simulink model "Modelado"  (R2023a)
settings: Solver=ode15s  StartTime=0.0  StopTime=15  MaxStep=1E-2  RelTol=1e-3
libraries: fl_lib x7, nesl_utility x3, slpidlib x2
settings Model: Creator=David  LastModifiedBy=David
settings DataIOCC: SaveOutput=off  SignalLogging=off  DSMLogging=off  ReturnWorkspaceOutputs=off  TimeSaveName=t
settings DebuggingCC: AlgebraicLoopMsg=none  ArtificialAlgebraicLoopMsg=none  MaxConsecutiveZCsMsg=none  ModelReferenceExtraNoncontSigs=none  OperatingPointInterfaceChecksumMismatchMsg=none
settings HardwareCC: ProdBitPerPointer=32  ProdBitPerSizeT=32  ProdBitPerPtrDiffT=32  ProdWordSize=32  ProdHWDeviceType=Intel->x86-32 (Windows32)

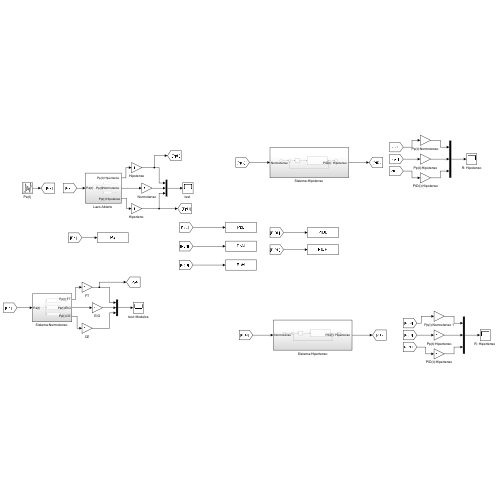
[thumbnail: Simulink's stored preview of the top-level diagram]
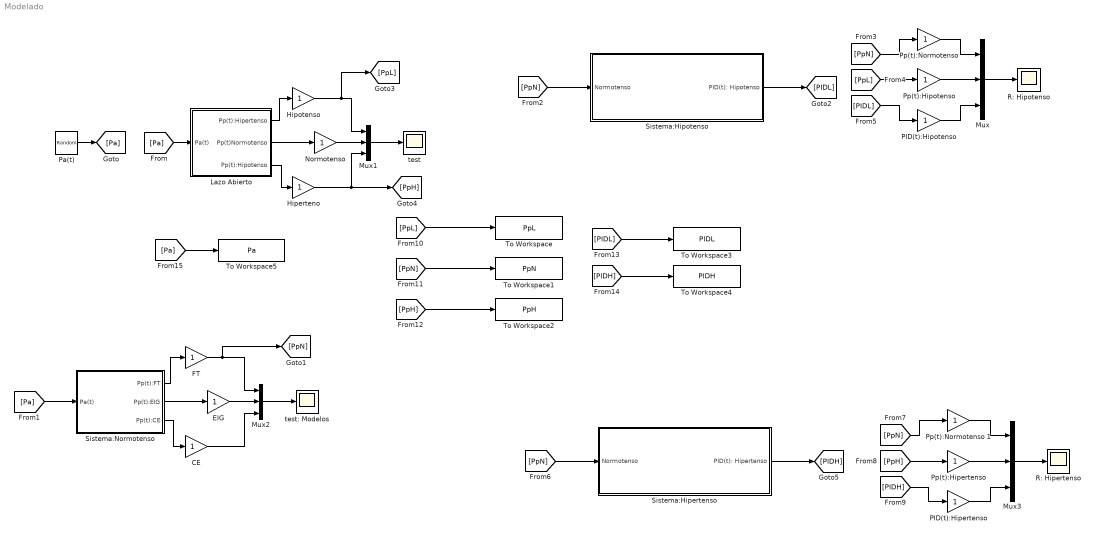
== system Modelado ==
  CE : Gain
  EIG : Gain
  FT : Gain
  "Hiperteno " : Gain
  Hipotenso : Gain
  "Lazo Abierto " : Subsystem
  Mux{,1..3} (4 alike) : Mux  Inputs=3
  Normotenso : Gain
  PID(t):Hipertenso : Gain
  PID(t):Hipotenso : Gain
  Pa(t) : UniformRandomNumber  Minimum=-0.2  Seed=106  SampleTime=0.1
  Pp(t):Hipertenso : Gain
  Pp(t):Hipotenso : Gain
  "Pp(t):Normotenso " : Gain
  Pp(t):Normotenso 1 : Gain
  "R: Hipertenso " : Scope
  R: Hipotenso : Scope
  Sistema:Hipertenso : Subsystem
  "Sistema:Hipotenso " : Subsystem
  "Sistema:Normotenso " : Subsystem
  To Workspace : ToWorkspace  VariableName=PpL  SampleTime=-1
  To Workspace1 : ToWorkspace  VariableName=PpN  SampleTime=-1
  To Workspace2 : ToWorkspace  VariableName=PpH  SampleTime=-1
  To Workspace3 : ToWorkspace  VariableName=PIDL  SampleTime=-1
  To Workspace4 : ToWorkspace  VariableName=PIDH  SampleTime=-1
  To Workspace5 : ToWorkspace  VariableName=Pa  SampleTime=-1
  "test " : Scope
  test: Modelos : Scope
  wires:
  Normotenso/1 -> Mux1/2
  "Lazo Abierto "/1("Pp(t):Hipertenso ") -> Hipotenso/1
  Hipotenso/1 -> [PpL], Mux1/1
  Pa(t)/1 -> [Pa]
  "Lazo Abierto "/2("Pp(t)Normotenso ") -> Normotenso/1
  "Lazo Abierto "/3(Pp(t):Hipotenso) -> "Hiperteno "/1
  [Pa] -> "Lazo Abierto "/1(Pa(t))
  Mux1/1 -> "test "/1
  "Sistema:Normotenso "/2(Pp(t):EIG) -> EIG/1
  FT/1 -> [PpN], Mux2/1
  Mux2/1 -> test: Modelos/1
  EIG/1 -> Mux2/2
  CE/1 -> Mux2/3
  "Sistema:Normotenso "/1(Pp(t):FT) -> FT/1
  "Sistema:Normotenso "/3(Pp(t):CE) -> CE/1
  [Pa] -> "Sistema:Normotenso "/1(Pa(t))
  [PpN] -> "Sistema:Hipotenso "/1("Normotenso ")
  "Sistema:Hipotenso "/1("PID(t): Hipotenso ") -> [PIDL]
  "Hiperteno "/1 -> [PpH], Mux1/3
  [PpN] -> "Pp(t):Normotenso "/1
  [PpL] -> Pp(t):Hipotenso/1
  [PIDL] -> PID(t):Hipotenso/1
  Mux/1 -> R: Hipotenso/1
  "Pp(t):Normotenso "/1 -> Mux/1
  Pp(t):Hipotenso/1 -> Mux/2
  PID(t):Hipotenso/1 -> Mux/3
  Sistema:Hipertenso/1("PID(t): Hipertenso ") -> [PIDH]
  [PpN] -> Sistema:Hipertenso/1("Normotenso ")
  [PpN] -> Pp(t):Normotenso 1/1
  Pp(t):Normotenso 1/1 -> Mux3/1
  PID(t):Hipertenso/1 -> Mux3/3
  Mux3/1 -> "R: Hipertenso "/1
  Pp(t):Hipertenso/1 -> Mux3/2
  [PIDH] -> PID(t):Hipertenso/1
  [PpH] -> Pp(t):Hipertenso/1
  [PpL] -> To Workspace/1
  [PpN] -> To Workspace1/1
  [PpH] -> To Workspace2/1
  [PIDL] -> To Workspace3/1
  [PIDH] -> To Workspace4/1
  [Pa] -> To Workspace5/1

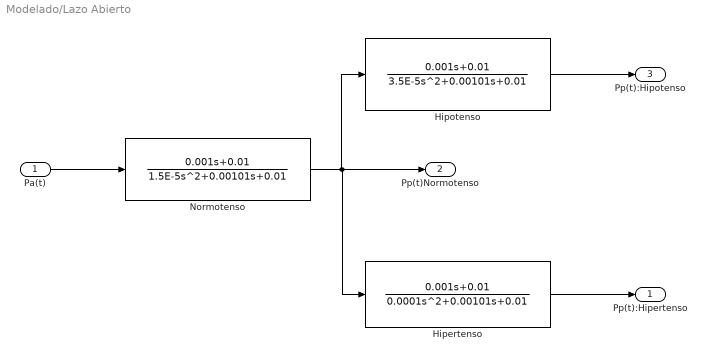
== system Modelado/Lazo Abierto  ==
  Pa(t) : Inport
  "Hipertenso " : TransferFcn  Numerator=[0.001, 0.01]  Denominator=[0.0001, 0.00101, 0.01]
  "Hipotenso " : TransferFcn  Numerator=[0.001, 0.01]  Denominator=[3.5E-5, 0.00101, 0.01]
  "Normotenso " : TransferFcn  Numerator=[0.001, 0.01]  Denominator=[1.5E-5, 0.00101, 0.01]
  "Pp(t):Hipertenso " : Outport
  "Pp(t)Normotenso " : Outport  Port=2
  Pp(t):Hipotenso : Outport  Port=3
  wires:
  Pa(t)/1 -> "Normotenso "/1
  "Normotenso "/1 -> "Hipotenso "/1, "Hipertenso "/1, "Pp(t)Normotenso "/1
  "Hipotenso "/1 -> Pp(t):Hipotenso/1
  "Hipertenso "/1 -> "Pp(t):Hipertenso "/1

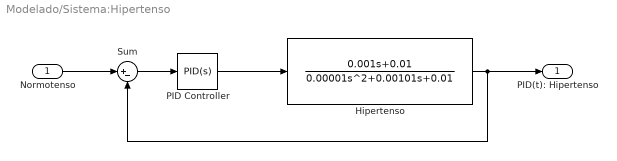
== system Modelado/Sistema:Hipertenso ==
  "Normotenso " : Inport
  "Hipertenso " : TransferFcn  Numerator=[0.001, 0.01]  Denominator=[0.00001, 0.00101, 0.01]
  PID Controller : slpidlib/PID Controller  Controller=PID  Form=Parallel  TimeDomain=Continuous-time  UseExternalTs=off  SampleTime=-1  IntegratorMethod=Forward Euler  FilterMethod=Forward Euler  ControllerParametersSource=internal  P=125.069829584559  I=289581.945280002  UseKiTs=off  D=0.00174354722386766  N=47733.2993032854  UseFilter=on  TunerSelectOption=Transfer Function Based (PID Tuner App)  InitialConditionSource=internal  InitialConditionForIntegrator=0  InitialConditionForFilter=0  DifferentiatorICPrevScaledInput=0  ExternalReset=none  TrackingMode=off  Kt=1  LimitOutput=off  SatLimitsSource=internal  UpperSaturationLimit=inf  LowerSaturationLimit=-inf  LinearizeAsGain=on  AntiWindupMode=none  Kb=1  LimitIntegrator=off  UpperIntegratorSaturationLimit=inf  LowerIntegratorSaturationLimit=-inf  POutMin=[]  POutMax=[]  IOutMin=[]  IOutMax=[]  DOutMin=[]  DOutMax=[]  NOutMin=[]  NOutMax=[]  SumOutMin=[]  SumOutMax=[]  SaturationOutMin=[]  SaturationOutMax=[]  PParamMin=[]  PParamMax=[]  IParamMin=[]  IParamMax=[]  DParamMin=[]  DParamMax=[]  NParamMin=[]  NParamMax=[]  KbParamMin=[]  KbParamMax=[]  KtParamMin=[]  KtParamMax=[]  KbOutMin=[]  KbOutMax=[]  KtOutMin=[]  KtOutMax=[]  IntegratorOutMin=[]  IntegratorOutMax=[]  FilterOutMin=[]  FilterOutMax=[]  SumI1OutMin=[]  SumI1OutMax=[]  SumI2OutMin=[]  SumI2OutMax=[]  SumI3OutMin=[]  SumI3OutMax=[]  SumI4OutMin=[]  SumI4OutMax=[]  SumDOutMin=[]  SumDOutMax=[]  DifferentiatorOutMin=[]  DifferentiatorOutMax=[]  FilterDiffOutCoefMin=[]  FilterDiffOutCoefMax=[]  ReciprocalOutMin=[]  ReciprocalOutMax=[]  SumDenOutMin=[]  SumDenOutMax=[]  SumNumOutMin=[]  SumNumOutMax=[]  DivideOutMin=[]  DivideOutMax=[]  UdiffTsProdOutMin=[]  UdiffTsProdOutMax=[]  NTsProdOutMin=[]  NTsProdOutMax=[]  UintegralTsProdOutMin=[]  UintegralTsProdOutMax=[]  UngainTsProdOutMin=[]  UngainTsProdOutMax=[]  ClampingZeroOutDataTypeStr=Inherit: Inherit via back propagation  ClampingZeroOutMin=[]  ClampingZeroOutMax=[]  FilterDenConstantOutDataTypeStr=Inherit: Inherit via back propagation  FilterDenConstantOutMin=[]  FilterDenConstantOutMax=[]  PCopyOutDataTypeStr=Inherit: Inherit via back propagation  PCopyOutMin=[]  PCopyOutMax=[]  NCopyOutDataTypeStr=Inherit: Inherit via back propagation  NCopyOutMin=[]  NCopyOutMax=[]  IntegratorContinuousStateAttributes=''  IntegratorStateMustResolveToSignalObject=off  IntegratorRTWStateStorageClass=Auto  FilterContinuousStateAttributes=''  FilterStateMustResolveToSignalObject=off  FilterRTWStateStorageClass=Auto  ParallelPVariant=InternalParameters  IdealPVariant=Disabled  IVariant=InternalParameters  DVariant=InternalParameters  IntegratorVariant=Continuous  SatVariant=Disabled  AWVariant=Passthrough  PCopyVariant=Disabled  TRVariant=Disabled  FdbkBlocksVariant=Forward  IdealPFdbkVariant=Disabled  SatFdbkVariant=Disabled  DerivativeFilterVariant=ContFilter  NVariant=InternalParameters  NCopyVariant=Disabled  FilterICVariant=InternalICsFilter  IntegratorICVariant=InternalICs  ExternalResetVariant=Disabled  TRSumVariant=Passthrough  SumFdbkVariant=Disabled  SumVariant=Sum_PID  TsampFilterVariant=InternalTs  TsampNgainVariant=Passthrough  TsampIntegralVariant=Disabled_SignalSpec  ExternalSaturationOutDataTypeStr=Inherit: Same as second input
  Sum : Sum  Inputs=|+-
  "PID(t): Hipertenso " : Outport
  wires:
  "Normotenso "/1 -> Sum/1
  Sum/1 -> PID Controller/1
  PID Controller/1 -> "Hipertenso "/1
  "Hipertenso "/1 -> "PID(t): Hipertenso "/1, Sum/2

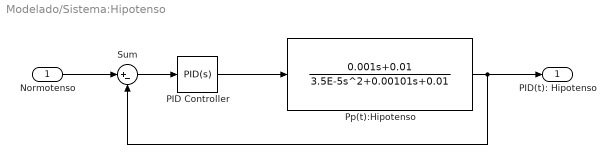
== system Modelado/Sistema:Hipotenso  ==
  "Normotenso " : Inport
  PID Controller : slpidlib/PID Controller  Controller=PID  Form=Parallel  TimeDomain=Continuous-time  UseExternalTs=off  SampleTime=-1  IntegratorMethod=Forward Euler  FilterMethod=Forward Euler  ControllerParametersSource=internal  P=458.48258315116  I=1112094.73550687  UseKiTs=off  D=0.00626713168710677  N=50057.6250783319  UseFilter=on  TunerSelectOption=Transfer Function Based (PID Tuner App)  InitialConditionSource=internal  InitialConditionForIntegrator=0  InitialConditionForFilter=0  DifferentiatorICPrevScaledInput=0  ExternalReset=none  TrackingMode=off  Kt=1  LimitOutput=off  SatLimitsSource=internal  UpperSaturationLimit=inf  LowerSaturationLimit=-inf  LinearizeAsGain=on  AntiWindupMode=none  Kb=1  LimitIntegrator=off  UpperIntegratorSaturationLimit=inf  LowerIntegratorSaturationLimit=-inf  POutMin=[]  POutMax=[]  IOutMin=[]  IOutMax=[]  DOutMin=[]  DOutMax=[]  NOutMin=[]  NOutMax=[]  SumOutMin=[]  SumOutMax=[]  SaturationOutMin=[]  SaturationOutMax=[]  PParamMin=[]  PParamMax=[]  IParamMin=[]  IParamMax=[]  DParamMin=[]  DParamMax=[]  NParamMin=[]  NParamMax=[]  KbParamMin=[]  KbParamMax=[]  KtParamMin=[]  KtParamMax=[]  KbOutMin=[]  KbOutMax=[]  KtOutMin=[]  KtOutMax=[]  IntegratorOutMin=[]  IntegratorOutMax=[]  FilterOutMin=[]  FilterOutMax=[]  SumI1OutMin=[]  SumI1OutMax=[]  SumI2OutMin=[]  SumI2OutMax=[]  SumI3OutMin=[]  SumI3OutMax=[]  SumI4OutMin=[]  SumI4OutMax=[]  SumDOutMin=[]  SumDOutMax=[]  DifferentiatorOutMin=[]  DifferentiatorOutMax=[]  FilterDiffOutCoefMin=[]  FilterDiffOutCoefMax=[]  ReciprocalOutMin=[]  ReciprocalOutMax=[]  SumDenOutMin=[]  SumDenOutMax=[]  SumNumOutMin=[]  SumNumOutMax=[]  DivideOutMin=[]  DivideOutMax=[]  UdiffTsProdOutMin=[]  UdiffTsProdOutMax=[]  NTsProdOutMin=[]  NTsProdOutMax=[]  UintegralTsProdOutMin=[]  UintegralTsProdOutMax=[]  UngainTsProdOutMin=[]  UngainTsProdOutMax=[]  ClampingZeroOutDataTypeStr=Inherit: Inherit via back propagation  ClampingZeroOutMin=[]  ClampingZeroOutMax=[]  FilterDenConstantOutDataTypeStr=Inherit: Inherit via back propagation  FilterDenConstantOutMin=[]  FilterDenConstantOutMax=[]  PCopyOutDataTypeStr=Inherit: Inherit via back propagation  PCopyOutMin=[]  PCopyOutMax=[]  NCopyOutDataTypeStr=Inherit: Inherit via back propagation  NCopyOutMin=[]  NCopyOutMax=[]  IntegratorContinuousStateAttributes=''  IntegratorStateMustResolveToSignalObject=off  IntegratorRTWStateStorageClass=Auto  FilterContinuousStateAttributes=''  FilterStateMustResolveToSignalObject=off  FilterRTWStateStorageClass=Auto  ParallelPVariant=InternalParameters  IdealPVariant=Disabled  IVariant=InternalParameters  DVariant=InternalParameters  IntegratorVariant=Continuous  SatVariant=Disabled  AWVariant=Passthrough  PCopyVariant=Disabled  TRVariant=Disabled  FdbkBlocksVariant=Forward  IdealPFdbkVariant=Disabled  SatFdbkVariant=Disabled  DerivativeFilterVariant=ContFilter  NVariant=InternalParameters  NCopyVariant=Disabled  FilterICVariant=InternalICsFilter  IntegratorICVariant=InternalICs  ExternalResetVariant=Disabled  TRSumVariant=Passthrough  SumFdbkVariant=Disabled  SumVariant=Sum_PID  TsampFilterVariant=InternalTs  TsampNgainVariant=Passthrough  TsampIntegralVariant=Disabled_SignalSpec  ExternalSaturationOutDataTypeStr=Inherit: Same as second input
  "Pp(t):Hipotenso " : TransferFcn  Numerator=[0.001, 0.01]  Denominator=[3.5E-5, 0.00101, 0.01]
  Sum : Sum  Inputs=|+-
  "PID(t): Hipotenso " : Outport
  wires:
  "Normotenso "/1 -> Sum/1
  Sum/1 -> PID Controller/1
  PID Controller/1 -> "Pp(t):Hipotenso "/1
  "Pp(t):Hipotenso "/1 -> "PID(t): Hipotenso "/1, Sum/2

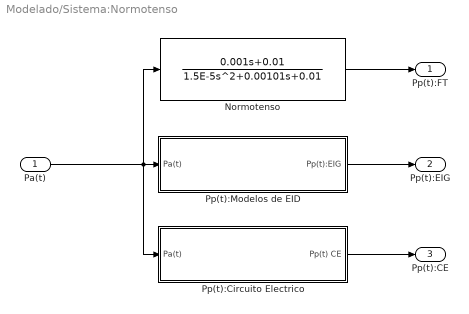
== system Modelado/Sistema:Normotenso  ==
  Pa(t) : Inport
  "Normotenso " : TransferFcn  Numerator=[0.001, 0.01]  Denominator=[1.5E-5, 0.00101, 0.01]
  "Pp(t):Circuito Electrico " : Subsystem
  Pp(t):Modelos de EID : Subsystem
  Pp(t):FT : Outport
  Pp(t):EIG : Outport  Port=2
  Pp(t):CE : Outport  Port=3
  wires:
  Pa(t)/1 -> "Pp(t):Circuito Electrico "/1(Pa(t)), "Normotenso "/1, Pp(t):Modelos de EID/1(Pa(t))
  Pp(t):Modelos de EID/1(Pp(t):EIG) -> Pp(t):EIG/1
  "Normotenso "/1 -> Pp(t):FT/1
  "Pp(t):Circuito Electrico "/1(Pp(t) CE) -> Pp(t):CE/1

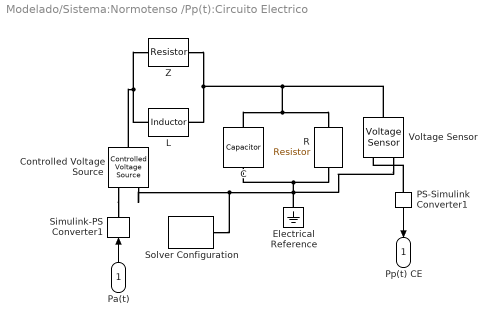
== system Modelado/Sistema:Normotenso /Pp(t):Circuito Electrico  ==
  Pa(t) : Inport
  C : fl_lib/Electrical/Electrical Elements/Capacitor  c=1.5 F  r=1e-6 Ohm  g=0 1/Ohm  i_specify=off  i_priority=None  i=0 A  i_nominal_specify=off  i_nominal_unit=A  i_nominal_value=1  v_specify=off  v_priority=None  v=0 V  v_nominal_specify=off  v_nominal_unit=V  v_nominal_value=1  vc_specify=off  vc_priority=High  vc=0 V  vc_nominal_specify=off  vc_nominal_unit=V  vc_nominal_value=1
  Controlled Voltage Source : fl_lib/Electrical/Electrical Sources/Controlled Voltage Source
  Electrical Reference : fl_lib/Electrical/Electrical Elements/Electrical Reference
  L : fl_lib/Electrical/Electrical Elements/Inductor  l=0.001 H  r=0 Ohm  g=1e-9 1/Ohm  i_specify=off  i_priority=None  i=0 A  i_nominal_specify=off  i_nominal_unit=A  i_nominal_value=1  v_specify=off  v_priority=None  v=0 V  v_nominal_specify=off  v_nominal_unit=V  v_nominal_value=1  i_L_specify=off  i_L_priority=High  i_L=0 A  i_L_nominal_specify=off  i_L_nominal_unit=A  i_L_nominal_value=1
  PS-Simulink Converter1 : nesl_utility/PS-Simulink Converter  PhysicalDomain=network_engine_domain  SubClassName=ps_output  LeftPortType=input  RightPortType=output  PseudoPeriodic=off  Frequencies=[]  VectorFormat=inherit  Unit=inherit  AffineConversion=off
  R : fl_lib/Electrical/Electrical Elements/Resistor  R=1 Ohm  i_specify=off  i_priority=None  i=0 A  i_nominal_specify=off  i_nominal_unit=A  i_nominal_value=1  v_specify=off  v_priority=None  v=0 V  v_nominal_specify=off  v_nominal_unit=V  v_nominal_value=1
  Simulink-PS Converter1 : nesl_utility/Simulink-PS Converter  PhysicalDomain=network_engine_domain  SubClassName=ps_input  LeftPortType=input  RightPortType=output  PseudoPeriodic=off  Frequencies=[]  NoiseDistribution=none  NoiseParameters=[]  Unit=1  AffineConversion=off  FilteringAndDerivatives=provide  SimscapeFilterOrder=1  InputFilterTimeConstant=0.001  UdotUserProvided=0
  Solver Configuration : nesl_utility/Solver Configuration  PhysicalDomain=network_engine_domain  SubClassName=solver  LeftPortType=input  RightPortType=generic  Tones=[]  Harmonics=[]  SimulateNoise=off  Profile=off  UseLocalSampling=off  EnableSwitchedLinearOptims=on  FrequencyDomain=off  UseCCode=off  RelTol=0.001  AbsTol=0.001  MinStep=1e-09  ToWorkspace=off  RevertToSquareIcSolve=off  NumHomotopyIterations=100  PhasorMode=off  PhasorModeNumHarmonics=1  ConsistencySolver=NEWTON_XTOL_AFTER_FTOL  IndexReductionMethod=DerivativeReplacement  DoDC=off  ResidualTolerance=1e-09  ConsistencyTolSource=GLOBAL  ConsistencyAbsTol=0.001  ConsistencyRelTol=0.001  ConsistencyTolFactor=0.001  UseLocalSolver=off  LocalSolverChoice=NE_BACKWARD_EULER_ADVANCER  ResolveIndetEquations=on  FunctionEvalNumThread=1  LocalSolverSampleTime=0.001  DoFixedCost=off  MaxNonlinIter=3  MaxModeIter=2  ComputeImpulses=off  ImpulseIterations=2  LinearAlgebra=auto  LinearAlgebraNumThread=0  EquationFormulation=NE_TIME_EF  DelaysMemoryBudget=1024  AutomaticFiltering=on  FilteringTimeConstant=0.001  PartitionStorageMethod=AS_NEEDED  PartitionMemoryBudget=1024  PartitionMethod=ROBUST
  Voltage Sensor : fl_lib/Electrical/Electrical Sensors/Voltage Sensor
  Z : fl_lib/Electrical/Electrical Elements/Resistor  R=0.010 Ohm  i_specify=off  i_priority=None  i=0 A  i_nominal_specify=off  i_nominal_unit=A  i_nominal_value=1  v_specify=off  v_priority=None  v=0 V  v_nominal_specify=off  v_nominal_unit=V  v_nominal_value=1
  Pp(t) CE : Outport
  wires:
  Pa(t)/1 -> Simulink-PS Converter1/1
  PS-Simulink Converter1/1 -> Pp(t) CE/1
  connections:
  L/LConn1 -- Z/LConn1 -- Controlled Voltage Source/LConn1
  Z/RConn1 -- Voltage Sensor/LConn1 -- R/LConn1 -- C/LConn1 -- L/RConn1
  R/RConn1 -- Solver Configuration/RConn1 -- Controlled Voltage Source/RConn2 -- Electrical Reference/LConn1 -- Voltage Sensor/RConn2 -- C/RConn1
  PS-Simulink Converter1/LConn1 -- Voltage Sensor/RConn1
  Controlled Voltage Source/RConn1 -- Simulink-PS Converter1/RConn1

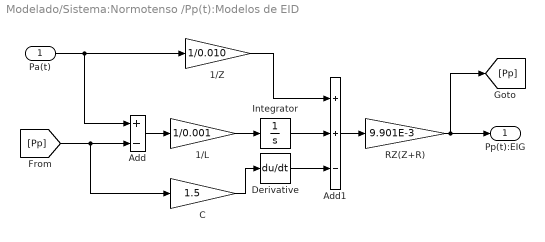
== system Modelado/Sistema:Normotenso /Pp(t):Modelos de EID ==
  Pa(t) : Inport
  1/L : Gain  Gain=1/0.001
  1/Z : Gain  Gain=1/0.010
  Add : Sum  Inputs=+-
  Add1 : Sum  Inputs=++-
  C : Gain  Gain=1.5
  Derivative : Derivative
  Integrator : Integrator
  RZ(Z+R) : Gain  Gain=9.901E-3
  Pp(t):EIG : Outport
  wires:
  Integrator/1 -> Add1/2
  Derivative/1 -> Add1/3
  1/Z/1 -> Add1/1
  Pa(t)/1 -> Add/1, 1/Z/1
  [Pp] -> C/1, Add/2
  Add/1 -> 1/L/1
  1/L/1 -> Integrator/1
  C/1 -> Derivative/1
  Add1/1 -> RZ(Z+R)/1
  RZ(Z+R)/1 -> Pp(t):EIG/1, [Pp]
